simulink model "Slip_Control_codegen"  (R2025b)
settings: Solver=FixedStepDiscrete  StartTime=0.0  StopTime=100  FixedStep=0.003  MaxStep=0.4  RelTol=1e-3  AbsTol=1e-3
model mask{Af=Af, Control=Control, Gr=Gr, L=L, Load_Ref=Load_Ref, MotorT=MotorT, MotorW=MotorW, Slip_Ref=Slip_Ref, Tmax=Tmax, a=a, a_cop=a_cop, cd=cd, g=g, h_CG=h_CG, m=m, ro=ro, rwheel=rwheel, tr=tr, vx_th=vx_th}
model workspace (MAT data in the model file):
  Af = 1.2
  Control.Name = 'SlipControl'
  Control.Steer.Gain.vVehicle.Value = [0 5.26315789474 10.5263157895 15.7894736842 21.0526315789 26.3157894737 31.5789473684 36.8421052632 42.1052631579 47.3684210526 52.6315789474 57.8947368421 63.1578947368 68.4210526316 73.6842105263 78.9473684211 84.2105263158 89.4736842105 94.7368421053 100 180]
  Control.Steer.Gain.vVehicle.Units = 'km/h'
  Control.Steer.Gain.n.Value = [0 -0.3 -0.299810360003 -0.279980668816 -0.23770520484 -0.184653739612 -0.080055401662 0.0617728531856 0.198282548476 0.286925207756 0.3 0.3 0.3 0.3 0.282374573553 0.212225572241 0.119402711766 0.037496894591 9.90231812217e-05 0 0]
  Control.Steer.fActuatorCutoff.Value = 50
  Control.Steer.fActuatorCutoff.Units = 'Hz'
  Control.Steer.Limits.aUpper.Value = 0.174532925199
  Control.Steer.Limits.aUpper.Units = 'rad'
  Control.Steer.Limits.aLower.Value = -0.174532925199
  Control.WheelRad = 0.263
  Control.GearRatio = 5
  Control.MotorTrq = [51.0306904762 51.0306904762 51.0306904762 51.0306904762 51.0306904762 51.0306904762 51.0306904762 51.0306904762 51.0306904762 51.0306904762 51.0306904762 51.0306904762 51.0306904762 51.0306904762 51.0306904762 51.0306904762 51.0306904762 51.0306904762 51.0306904762 51.0306904762 51.0306904762 51.0306904762 51.0306904762 51.0306904762 51.0306904762 51.0306904762 51.0306904762 51.0306904762 51.0306904762 51.0306904762 51.0306904762 51.0306904762 51.0306904762 51.0306904762 51.0306904762 51.0306904762 51.0306904762 44.8436898333 36.8215688219 30.0627288241 25.3370743141 21.0374123095 17.0840324268 13.4184887499 9.99592684833 6.77696534591 3.73957484604]
  Control.MotorW = [0 100 200 300 400 500 600 700 800 900 1000 1100 1200 1300 1400 1500 1600 1700 1800 1900 2000 2100 2200 2300 2400 2500 2600 2700 2800 2900 3000 3100 3200 3300 3400 3500 3600 3700 3800 3900 4000 4100 4200 4300 4400 4500 4600]
  Control.Tmax = 51.0306904762
  Control.RearTrack = 1.248
  Control.FrontTrackToCG = 0.823
  Control.FrontTrackToCoP = 0.8
  Control.FrontalArea = 1.2
  Control.Proportional_P = 1550
  Control.Integral_I = 38025
  Control.Derivative_D = 8
  Control.ActivationVelocity = 0.7
  Control.LiftCoef = -2.15
  Control.GravitationAcc = 9.81
  Control.CGHeight = 0.315
  Control.Wheelbase = 1.575
  Control.Mass = 315
  Control.AirDensity = 1.226
  Control.SlipRef = [0.08; 0.08; 0.152; 0.116; 0.102; 0.096; 0.092; 0.09; 0.09; 0.09; 0.094; 0.098; 0.104; 0.112; 0.126; 0.154; 0.232; 0.1]
  Control.LoadRef = [0; 400; 500; 600; 700; 800; 900; 1000; 1100; 1200; 1300; 1400; 1500; 1600; 1700; 1800; 1900; 2000]
  Gr = 5
  L = 1.578
  Load_Ref = [0; 400; 500; 600; 700; 800; 900; 1000; 1100; 1200; 1300; 1400; 1500; 1600; 1700; 1800; 1900; 2000]
  MotorT = [51.0306904762 51.0306904762 51.0306904762 51.0306904762 51.0306904762 51.0306904762 51.0306904762 51.0306904762 51.0306904762 51.0306904762 51.0306904762 51.0306904762 51.0306904762 51.0306904762 51.0306904762 51.0306904762 51.0306904762 51.0306904762 51.0306904762 51.0306904762 51.0306904762 51.0306904762 51.0306904762 51.0306904762 51.0306904762 51.0306904762 51.0306904762 51.0306904762 51.0306904762 51.0306904762 51.0306904762 51.0306904762 51.0306904762 51.0306904762 51.0306904762 51.0306904762 51.0306904762 44.8436898333 36.8215688219 30.0627288241 25.3370743141 21.0374123095 17.0840324268 13.4184887499 9.99592684833 6.77696534591 3.73957484604]
  MotorW = [0 100 200 300 400 500 600 700 800 900 1000 1100 1200 1300 1400 1500 1600 1700 1800 1900 2000 2100 2200 2300 2400 2500 2600 2700 2800 2900 3000 3100 3200 3300 3400 3500 3600 3700 3800 3900 4000 4100 4200 4300 4400 4500 4600]
  Slip_Ctrl_Kd = Simulink.Parameter
  Slip_Ctrl_Kd.Value = 11
  Slip_Ctrl_Kd.Complexity = 'real'
  Slip_Ctrl_Kd.Dimensions = [1 1]
  Slip_Ctrl_Kd.CoderInfo.StorageClass = 'ImportedExtern'
  Slip_Ctrl_Kd.DataType = 'single'
  Slip_Ctrl_Ki = Simulink.Parameter
  Slip_Ctrl_Ki.Value = 6000
  Slip_Ctrl_Ki.Complexity = 'real'
  Slip_Ctrl_Ki.Dimensions = [1 1]
  Slip_Ctrl_Ki.CoderInfo.StorageClass = 'ImportedExtern'
  Slip_Ctrl_Ki.DataType = 'single'
  Slip_Ctrl_Kn = Simulink.Parameter
  Slip_Ctrl_Kn.Value = 100
  Slip_Ctrl_Kn.Complexity = 'real'
  Slip_Ctrl_Kn.Dimensions = [1 1]
  Slip_Ctrl_Kn.CoderInfo.StorageClass = 'ImportedExtern'
  Slip_Ctrl_Kn.DataType = 'single'
  Slip_Ctrl_Kp = Simulink.Parameter
  Slip_Ctrl_Kp.Value = 800
  Slip_Ctrl_Kp.Complexity = 'real'
  Slip_Ctrl_Kp.Dimensions = [1 1]
  Slip_Ctrl_Kp.CoderInfo.StorageClass = 'ImportedExtern'
  Slip_Ctrl_Kp.DataType = 'single'
  Slip_Ref = [0.08; 0.08; 0.09; 0.095; 0.093; 0.092; 0.091; 0.09; 0.09; 0.09; 0.094; 0.098; 0.104; 0.112; 0.126; 0.154; 0.2; 0.12]
  Tmax = 51.0306904762
  a = 0.8232
  a_cop = 0.707
  cd = -2.15
  g = 9.81
  h_CG = 0.3583
  m = 320
  ro = 1.226
  rwheel = 0.263
  tr = 1.25
  vx_th = 0.7
undefined symbols (not defined in the file or in its folder): dspblkCoreblockFVToolHelper, gcbh
libraries: slpidlib x2
settings Model: TunableVars=Kp  TunableVarsStorageClass=ExportedGlobal  TunableVarsTypeQualifier=const  ParameterArgumentNames=Af,Control,Gr,L,Load_Ref,MotorT,MotorW,Slip_Ref,Tmax,a,a_cop,cd,g,h_CG,m,ro,rwheel,tr,vx_th  Creator=smiller  LastModifiedBy=andrei
settings SolverCC: MaxConsecutiveMinStep=5  AlgebraicLoopSolver=TrustRegion  AutoInsertRateTranBlk=on  InsertRTBMode=Never (minimum delay)  MinimalZcImpactIntegration=on
settings DataIOCC: MaxDataPoints=10000  SaveFormat=StructureWithTime  SaveOutput=off  SignalLogging=off  DSMLogging=off  SaveTime=off  ReturnWorkspaceOutputs=off  SignalLoggingName=logsout_sm_car
settings OptimizationCC: DefaultParameterBehavior=Inlined  UseDivisionForNetSlopeComputation=on  GainParamInheritBuiltInType=on  UseFloatMulNetSlope=on  DefaultUnderspecifiedDataType=single  UseSpecifiedMinMax=on  PassReuseOutputArgsAs=Individual arguments  NoFixptDivByZeroProtection=on  EfficientFloat2IntCast=on  LifeSpan=inf  OptimizeBlockOrder=speed  DifferentSizesBufferReuse=on  EfficientTunableParamExpr=on
settings DebuggingCC: ReadBeforeWriteMsg=EnableAllAsError  WriteAfterWriteMsg=EnableAllAsError  WriteAfterReadMsg=EnableAllAsError  AlgebraicLoopMsg=none  IntegerOverflowMsg=error  ParameterPrecisionLossMsg=none  ParameterTunabilityLossMsg=error  UnconnectedInputMsg=warning  UnconnectedOutputMsg=warning  UnconnectedLineMsg=warning  UniqueDataStoreMsg=error  NonBusSignalsTreatedAsBus=error  SFInvalidInputDataAccessInChartInitDiag=error  SFTransitionOutsideNaturalParentDiag=error  SFUnreachableExecutionPathDiag=error  SFUndirectedBroadcastEventsDiag=error  IntegerSaturationMsg=error  ArithmeticOperatorsInVariantConditions=warning
settings HardwareCC: ProdBitPerPointer=32.0  ProdBitPerSizeT=32.0  ProdBitPerPtrDiffT=32.0  ProdLargestAtomicInteger=Long  ProdLargestAtomicFloat=Double  ProdWordSize=32.0  ProdHWDeviceType=ARM Compatible->ARM Cortex-M
settings ModelReferenceCC: EnableRefExpFcnMdlSchedulingChecks=on
settings SFSimCC: MATLABDynamicMemAlloc=off  CustomCodeUndefinedFunction=UseInterfaceOnly
settings RTWCC: SystemTargetFile=ert.tlc  TemplateMakefile=ert_default_tmf  BuildConfiguration=Faster Runs  GPUComputeCapability=3.5  DLArmComputeVersion=19.05  Description=Embedded Coder
settings CodeAppCC: ForceParamTrailComments=on  IgnoreCustomStorageClasses=off  OperatorAnnotations=on  SimulinkDataObjDesc=on  SFDataObjDesc=on  CustomSymbolStrGlobalVar=rt$N$M  CustomSymbolStrType=$N$M  CustomSymbolStrFcn=$N$M$F  CustomSymbolStrMacro=$N$M  InsertBlockDesc=on
settings ERTTargetCC: ERTCustomFileTemplate=example_file_process.tlc  ERTFilePackagingFormat=CompactWithDataFile  GenerateSampleERTMain=on  IncludeMdlTerminateFcn=off  CombineSignalStateStructs=on  SuppressErrorStatus=on  SupportAbsoluteTime=off  CodeInterfacePackaging=Reusable function  SupportComplex=off
settings SimscapeCC: SimscapeLogType=all  SimscapeLogSimulationStatistics=on  SimscapeLogName=simlog_sm_car  SimscapeLogDataHistory=100000.0  SimscapeOperatingPoint=ssc_op
settings DiagnosticsConfigSet: SimMechanicsConflictingReferenceFrames=none  SimMechanicsRigidlyBoundBlock=none  SimMechanicsUnsatisfiedHighPriorityTargets=error
settings ExplorerConfigSet: InternalSimMechanicsExplorerSettings="<ExplorerConfiguration><canonicalview>default</canonicalview><AnimationSetting><BasePlaybackSpeed>1.0</BasePlaybackSpeed><PlaybackSpeedFactor>1.0</PlaybackSpeedFactor></AnimationSetting><TilePanel><TileInfo><Tiles Columns=\"1\" Count=\"1\" Rows=\"1\"><Column Weight=\"1\"/><Row Weight=\"1\"/><Tile Height=\"1\" Width=\"1\" X=\"0\" Y=\"0\"/></Tiles></TileInfo><SceneInfo><SceneViewer><BGColor><R>1</R><G>1</G><B>1</B></BGColor><Camera><DoPerspective>on</DoPerspective><Position><X>-22.5734563329168161</X><Y>-2.56079992530625722</Y><Z>1.4393604008155032</Z></Position><Center><X>-23.2962680852000119</X><Y>-1.95845679840359432</Y><Z>1.10064823948317181</Z></Center><Up><X>-0.260205889993916473</X><Y>0.216838241661597014</Y><Z>0.940890042335224552</Z></Up><ViewLimDist>1</ViewLimDist><YLim>0.466307658154998694</YLim><XLim>0.489818968650208741</XLim></Camera></SceneViewer></SceneInfo></TilePanel><MechEditorPanel><Cameras><Camera><Id>Camera1</Id><Value><Name>Track FixO FR</Name><NativeCamera><PositionTrackingFeature>Camera_Frames.Frame_FixO_FR.R</PositionTrackingFeature><CenterTrackingFeature>Camera_Frames.Frame_FixO_FR.R</CenterTrackingFeature><UpVectorTrackingFeature>Camera_Frames.Frame_FixO_FR.R</UpVectorTrackingFeature><CenterTrackingOrigin>off</CenterTrackingOrigin><CenterTrackingDirection>+X</CenterTrackingDirection><UpVectorTrackingDirection>+Z</UpVectorTrackingDirection></NativeCamera></Value></Camera><Camera><Id>Camera2</Id><Value><Name>Track FixO Right</Name><NativeCamera><PositionTrackingFeature>Camera_Frames.Frame_FixO_Right.R</PositionTrackingFeature><CenterTrackingFeature>Camera_Frames.Transform_Camera_Ref.F</CenterTrackingFeature><UpVectorTrackingFeature>Camera_Frames.Frame_FixO_Right.R</UpVectorTrackingFeature><CenterTrackingOrigin>off</CenterTrackingOrigin><CenterTrackingDirection>+Y</CenterTrackingDirection><UpVectorTrackingDirection>+Z</UpVectorTrackingDirection></NativeCamera></Value></Camera><Camera><Id>Camera3</Id><Value><Name>Track FixO RR</Name><NativeCamera><PositionTrackingFeature>Camera_Frames.Frame_FixO_RR.R</PositionTrackingFeature><CenterTrackingFeature>Camera_Frames.Frame_FixO_RR.R</CenterTrackingFeature><UpVectorTrackingFeature>Camera_Frames.Frame_FixO_RR.R</UpVectorTrackingFeature><CenterTrackingOrigin>off</CenterTrackingOrigin><CenterTrackingDirection>+X</CenterTrackingDirection><UpVectorTrackingDirection>+Z</UpVectorTrackingDirection></NativeCamera></Value></Camera><Camera><Id>Camera4</Id><Value><Name>Track FixO RL</Name><NativeCamera><PositionTrackingFeature>Camera_Frames.Frame_FixO_RL.R</PositionTrackingFeature><CenterTrackingFeature>Camera_Frames.Frame_FixO_RL.R</CenterTrackingFeature><UpVectorTrackingFeature>Camera_Frames.Frame_FixO_RL.R</UpVectorTrackingFeature><CenterTrackingOrigin>off</CenterTrackingOrigin><CenterTrackingDirection>+X</CenterTrackingDirection><UpVectorTrackingDirection>+Z</UpVectorTrackingDirection></NativeCamera></Value></Camera><Camera><Id>Camera5</Id><Value><Name>Track FixO Left</Name><NativeCamera><PositionTrackingFeature>Camera_Frames.Frame_FixO_Left.R</PositionTrackingFeature><CenterTrackingFeature>Camera_Frames.Transform_Camera_Ref.F</CenterTrackingFeature><UpVectorTrackingFeature>Camera_Frames.Frame_FixO_Left.R</UpVectorTrackingFeature><CenterTrackingOrigin>off</CenterTrackingOrigin><CenterTrackingDirection>-Y</CenterTrackingDirection><UpVectorTrackingDirection>+Z</UpVectorTrackingDirection></NativeCamera></Value></Camera><Camera><Id>Camera6</Id><Value><Name>Track FixO FL</Name><NativeCamera><PositionTrackingFeature>Camera_Frames.Frame_FixO_FL.R</PositionTrackingFeature><CenterTrackingFeature>Camera_Frames.Frame_FixO_FL.R</CenterTrackingFeature><UpVectorTrackingFeature>Camera_Frames.Frame_FixO_FL.R</UpVectorTrackingFeature><CenterTrackingOrigin>off</CenterTrackingOrigin><CenterTrackingDirection>+X</CenterTrackingDirection><UpVectorTrackingDirection>+Z</UpVectorTrackingDirection></NativeCamera></Value></Camera><Camera><Id>Camera7</Id><Value><Name>Track FixO Top</Name><NativeCamera><PositionTrackingFeature>Camera_Frames.Frame_FixO_Top.R</PositionTrackingFeature><CenterTrackingFeature>Camera_Frames.Frame_FixO_Top.R</CenterTrackingFeature><UpVectorTrackingFeature>Camera_Frames.Frame_FixO_Top.R</UpVectorTrackingFeature><CenterTrackingOrigin>off</CenterTrackingOrigin><CenterTrackingDirection>+X</CenterTrackingDirection><UpVectorTrackingDirection>+Z</UpVectorTrackingDirection></NativeCamera></Value></Camera><Camera><Id>Camera8</Id><Value><Name>Track FixO Front</Name><NativeCamera><PositionTrackingFeature>Camera_Frames.Frame_FixO_Front.R</PositionTrackingFeature><CenterTrackingFeature>Camera_Frames.Frame_FixO_Front.R</CenterTrackingFeature><UpVectorTrackingFeature>Camera_Frames.Frame_FixO_Front.R</UpVectorTrackingFeature><CenterTrackingOrigin>off</CenterTrackingOrigin><CenterTrackingDirection>+X</CenterTrackingDirection><UpVectorTrackingDirection>+Z</UpVectorTrackingDirection></NativeCamera></Value></Camera><Camera><Id>Camera9</Id><Value><Name>Track FixO Rear</Name><NativeCamera><PositionTrackingFeature>Camera_Frames.Frame_FixO_Rear.R</PositionTrackingFeature><CenterTrackingFeature>Camera_Frames.Frame_FixO_Rear.R</CenterTrackingFeature><UpVectorTrackingFeature>Camera_Frames.Frame_FixO_Rear.R</UpVectorTrackingFeature><CenterTrackingOrigin>off</CenterTrackingOrigin><CenterTrackingDirection>+X</CenterTrackingDirection><UpVectorTrackingDirection>+Z</UpVectorTrackingDirection></NativeCamera></Value></Camera><Camera><Id>Camera10</Id><Value><Name>Track FR</Name><NativeCamera><PositionTrackingFeature>Camera_Frames.Frame_FR.R</PositionTrackingFeature><CenterTrackingFeature>Camera_Frames.Frame_FR.R</CenterTrackingFeature><UpVectorTrackingFeature>Camera_Frames.Frame_FR.R</UpVectorTrackingFeature><CenterTrackingOrigin>off</CenterTrackingOrigin><CenterTrackingDirection>+X</CenterTrackingDirection><UpVectorTrackingDirection>+Z</UpVectorTrackingDirection></NativeCamera></Value></Camera><Camera><Id>Camera11</Id><Value><Name>Track Right</Name><NativeCamera><PositionTrackingFeature>Camera_Frames.Frame_Right.R</PositionTrackingFeature><CenterTrackingFeature>Camera_Frames.Transform_Camera_Ref.F</CenterTrackingFeature><UpVectorTrackingFeature>Camera_Frames.Frame_Right.R</UpVectorTrackingFeature><CenterTrackingOrigin>off</CenterTrackingOrigin><CenterTrackingDirection>+Y</CenterTrackingDirection><UpVectorTrackingDirection>+Z</UpVectorTrackingDirection></NativeCamera></Value></Camera><Camera><Id>Camera12</Id><Value><Name>Track RR</Name><NativeCamera><PositionTrackingFeature>Camera_Frames.Frame_RR.R</PositionTrackingFeature><CenterTrackingFeature>Camera_Frames.Frame_RR.R</CenterTrackingFeature><UpVectorTrackingFeature>Camera_Frames.Frame_RR.R</UpVectorTrackingFeature><CenterTrackingOrigin>off</CenterTrackingOrigin><CenterTrackingDirection>+X</CenterTrackingDirection><UpVectorTrackingDirection>+Z</UpVectorTrackingDirection></NativeCamera></Value></Camera><Camera><Id>Camera13</Id><Value><Name>Track RL</Name><NativeCamera><PositionTrackingFeature>Camera_Frames.Frame_RL.R</PositionTrackingFeature><CenterTrackingFeature>Camera_Frames.Frame_RL.R</CenterTrackingFeature><UpVectorTrackingFeature>Camera_Frames.Frame_RL.R</UpVectorTrackingFeature><CenterTrackingOrigin>off</CenterTrackingOrigin><CenterTrackingDirection>+X</CenterTrackingDirection><UpVectorTrackingDirection>+Z</UpVectorTrackingDirection></NativeCamera></Value></Camera><Camera><Id>Camera14</Id><Value><Name>Track Left</Name><NativeCamera><PositionTrackingFeature>Camera_Frames.Frame_Left.R</PositionTrackingFeature><CenterTrackingFeature>Camera_Frames.Transform_Camera_Ref.F</CenterTrackingFeature><UpVectorTrackingFeature>Camera_Frames.Frame_Left.R</UpVectorTrackingFeature><CenterTrackingOrigin>off</CenterTrackingOrigin><CenterTrackingDirection>-Y</CenterTrackingDirection><UpVectorTrackingDirection>+Z</UpVectorTrackingDirection></NativeCamera></Value></Camera><Camera><Id>Camera15</Id><Value><Name>Track FL</Name><NativeCamera><PositionTrackingFeature>Camera_Frames.Frame_FL.R</PositionTrackingFeature><CenterTrackingFeature>Camera_Frames.Frame_FL.R</CenterTrackingFeature><UpVectorTrackingFeature>Camera_Frames.Frame_FL.R</UpVectorTrackingFeature><CenterTrackingOrigin>off</CenterTrackingOrigin><CenterTrackingDirection>+X</CenterTrackingDirection><UpVectorTrackingDirection>+Z</UpVectorTrackingDirection></NativeCamera></Value></Camera><Camera><Id>Camera16</Id><Value><Name>Track Top</Name><NativeCamera><PositionTrackingFeature>Camera_Frames.Frame_Top.R</PositionTrackingFeature><CenterTrackingFeature>Camera_Frames.Frame_Top.R</CenterTrackingFeature><UpVectorTrackingFeature>Camera_Frames.Frame_Top.R</UpVectorTrackingFeature><CenterTrackingOrigin>off</CenterTrackingOrigin><CenterTrackingDirection>+X</CenterTrackingDirection><UpVectorTrackingDirection>+Z</UpVectorTrackingDirection></NativeCamera></Value></Camera><Camera><Id>Camera17</Id><Value><Name>Track Front</Name><NativeCamera><PositionTrackingFeature>Camera_Frames.Frame_Front.R</PositionTrackingFeature><CenterTrackingFeature>Camera_Frames.Frame_Front.R</CenterTrackingFeature><UpVectorTrackingFeature>Camera_Frames.Frame_Front.R</UpVectorTrackingFeature><CenterTrackingOrigin>off</CenterTrackingOrigin><CenterTrackingDirection>+X</CenterTrackingDirection><UpVectorTrackingDirection>+Z</UpVectorTrackingDirection></NativeCamera></Value></Camera><Camera><Id>Camera18</Id><Value><Name>Track Rear</Name><NativeCamera><PositionTrackingFeature>Camera_Frames.Frame_Rear.R</PositionTrackingFeature><CenterTrackingFeature>Camera_Frames.Frame_Rear.R</CenterTrackingFeature><UpVectorTrackingFeature>Camera_Frames.Frame_Rear.R</UpVectorTrackingFeature><CenterTrackingOrigin>off</CenterTrackingOrigin><CenterTrackingDirection>+X</CenterTrackingDirection><UpVectorTrackingDirection>+Z</UpVectorTrackingDirection></NativeCamera></Value></Camera><Camera><Id>Camera19</Id><Value><Name>Track SuspF</Name><NativeCamera><PositionTrackingFeature>Camera_Frames.Frame_SuspF.R</PositionTrackingFeature><CenterTrackingFeature>Camera_Frames.Frame_SuspF.R</CenterTrackingFeature><UpVectorTrackingFeature>Camera_Frames.Frame_SuspF.R</UpVectorTrackingFeature><CenterTrackingOrigin>off</CenterTrackingOrigin><CenterTrackingDirection>+X</CenterTrackingDirection><UpVectorTrackingDirection>+Z</UpVectorTrackingDirection></NativeCamera></Value></Camera><Camera><Id>Camera20</Id><Value><Name>Track SuspR</Name><NativeCamera><PositionTrackingFeature>Camera_Frames.Frame_SuspR.R</PositionTrackingFeature><CenterTrackingFeature>Camera_Frames.Frame_SuspR.R</CenterTrackingFeature><UpVectorTrackingFeature>Camera_Frames.Frame_SuspR.R</UpVectorTrackingFeature><CenterTrackingOrigin>off</CenterTrackingOrigin><CenterTrackingDirection>+X</CenterTrackingDirection><UpVectorTrackingDirection>+Z</UpVectorTrackingDirection></NativeCamera></Value></Camera><Camera><Id>Camera21</Id><Value><Name>Track WheelFR</Name><NativeCamera><PositionTrackingFeature>Camera_Frames.Frame_Wheel_FR.R</PositionTrackingFeature><CenterTrackingFeature>Camera_Frames.Frame_Wheel_FR.R</CenterTrackingFeature><UpVectorTrackingFeature>Camera_Frames.Frame_Wheel_FR.R</UpVectorTrackingFeature><CenterTrackingOrigin>off</CenterTrackingOrigin><CenterTrackingDirection>+X</CenterTrackingDirection><UpVectorTrackingDirection>+Z</UpVectorTrackingDirection></NativeCamera></Value></Camera><Camera><Id>Camera22</Id><Value><Name>Track WheelRR</Name><NativeCamera><PositionTrackingFeature>Camera_Frames.Frame_Wheel_RR.R</PositionTrackingFeature><CenterTrackingFeature>Camera_Frames.Frame_Wheel_RR.R</CenterTrackingFeature><UpVectorTrackingFeature>Camera_Frames.Frame_Wheel_RR.R</UpVectorTrackingFeature><CenterTrackingOrigin>off</CenterTrackingOrigin><CenterTrackingDirection>+X</CenterTrackingDirection><UpVectorTrackingDirection>+Z</UpVectorTrackingDirection></NativeCamera></Value></Camera><Camera><Id>Camera23</Id><Value><Name>Track WheelRL</Name><NativeCamera><PositionTrackingFeature>Camera_Frames.Frame_Wheel_RL.R</PositionTrackingFeature><CenterTrackingFeature>Camera_Frames.Frame_Wheel_RL.R</CenterTrackingFeature><UpVectorTrackingFeature>Camera_Frames.Frame_Wheel_RL.R</UpVectorTrackingFeature><CenterTrackingOrigin>off</CenterTrackingOrigin><CenterTrackingDirection>+X</CenterTrackingDirection><UpVectorTrackingDirection>+Z</UpVectorTrackingDirection></NativeCamera></Value></Camera><Camera><Id>Camera24</Id><Value><Name>Track WheelFL</Name><NativeCamera><PositionTrackingFeature>Camera_Frames.Frame_Wheel_FL.R</PositionTrackingFeature><CenterTrackingFeature>Camera_Frames.Frame_Wheel_FL.R</CenterTrackingFeature><UpVectorTrackingFeature>Camera_Frames.Frame_Wheel_FL.R</UpVectorTrackingFeature><CenterTrackingOrigin>off</CenterTrackingOrigin><CenterTrackingDirection>+X</CenterTrackingDirection><UpVectorTrackingDirection>+Z</UpVectorTrackingDirection></NativeCamera></Value></Camera><Camera><Id>Camera25</Id><Value><Name>View Seat FL</Name><NativeCamera><PositionTrackingFeature>Camera_Frames.Frame_View_Seat_FL.R</PositionTrackingFeature><CenterTrackingFeature>Camera_Frames.Frame_View_Seat_FL.R</CenterTrackingFeature><UpVectorTrackingFeature>Camera_Frames.Frame_View_Seat_FL.R</UpVectorTrackingFeature><CenterTrackingOrigin>off</CenterTrackingOrigin><CenterTrackingDirection>+X</CenterTrackingDirection><UpVectorTrackingDirection>+Z</UpVectorTrackingDirection></NativeCamera></Value></Camera><Camera><Id>Camera26</Id><Value><Name>View Seat FR</Name><NativeCamera><PositionTrackingFeature>Camera_Frames.Frame_View_Seat_FR.R</PositionTrackingFeature><CenterTrackingFeature>Camera_Frames.Frame_View_Seat_FR.R</CenterTrackingFeature><UpVectorTrackingFeature>Camera_Frames.Frame_View_Seat_FR.R</UpVectorTrackingFeature><CenterTrackingOrigin>off</CenterTrackingOrigin><CenterTrackingDirection>+X</CenterTrackingDirection><UpVectorTrackingDirection>+Z</UpVectorTrackingDirection></NativeCamera></Value></Camera><Camera><Id>Camera27</Id><Value><Name>View Susp FR</Name><NativeCamera><PositionTrackingFeature>Camera_Frames.Frame_View_Susp_FR.R</PositionTrackingFeature><CenterTrackingFeature>Camera_Frames.Frame_View_Susp_FR.R</CenterTrackingFeature><UpVectorTrackingFeature>Camera_Frames.Frame_View_Susp_FR.R</UpVectorTrackingFeature><CenterTrackingOrigin>off</CenterTrackingOrigin><CenterTrackingDirection>+X</CenterTrackingDirection><UpVectorTrackingDirection>+Z</UpVectorTrackingDirection></NativeCamera></Value></Camera><Camera><Id>Camera28</Id><Value><Name>View Susp RR</Name><NativeCamera><PositionTrackingFeature>Camera_Frames.Frame_View_Susp_RR.R</PositionTrackingFeature><CenterTrackingFeature>Camera_Frames.Frame_View_Susp_RR.R</CenterTrackingFeature><UpVectorTrackingFeature>Camera_Frames.Frame_View_Susp_RR.R</UpVectorTrackingFeature><CenterTrackingOrigin>off</CenterTrackingOrigin><CenterTrackingDirection>+X</CenterTrackingDirection><UpVectorTrackingDirection>+Z</UpVectorTrackingDirection></NativeCamera></Value></Camera><Camera><Id>Camera29</Id><Value><Name>View Susp RL</Name><NativeCamera><PositionTrackingFeature>Camera_Frames.Frame_View_Susp_RL.R</PositionTrackingFeature><CenterTrackingFeature>Camera_Frames.Frame_View_Susp_RL.R</CenterTrackingFeature><UpVectorTrackingFeature>Camera_Frames.Frame_View_Susp_RL.R</UpVectorTrackingFeature><CenterTrackingOrigin>off</CenterTrackingOrigin><CenterTrackingDirection>+X</CenterTrackingDirection><UpVectorTrackingDirection>+Z</UpVectorTrackingDirection></NativeCamera></Value></Camera><Camera><Id>Camera30</Id><Value><Name>View Susp FL</Name><NativeCamera><PositionTrackingFeature>Camera_Frames.Frame_View_Susp_FL.R</PositionTrackingFeature><CenterTrackingFeature>Camera_Frames.Frame_View_Susp_FL.R</CenterTrackingFeature><UpVectorTrackingFeature>Camera_Frames.Frame_View_Susp_FL.R</UpVectorTrackingFeature><CenterTrackingOrigin>off</CenterTrackingOrigin><CenterTrackingDirection>+X</CenterTrackingDirection><UpVectorTrackingDirection>+Z</UpVectorTrackingDirection></NativeCamera></Value></Camera><Camera><Id>Camera31</Id><Value><Name>Dolly Camera</Name><NativeCamera><PositionTrackingFeature>Camera_Frames.Frame_Dolly.R</PositionTrackingFeature><CenterTrackingFeature>Camera_Frames.Frame_Dolly.R</CenterTrackingFeature><UpVectorTrackingFeature>Camera_Frames.Frame_Dolly.R</UpVectorTrackingFeature><CenterTrackingOrigin>off</CenterTrackingOrigin><CenterTrackingDirection>+X</CenterTrackingDirection><UpVectorTrackingDirection>+Z</UpVectorTrackingDirection></NativeCamera></Value></Camera><Camera><Id>Camera32</Id><Value><Name>Track Dolly Camera</Name><NativeCamera><PositionTrackingFeature>Camera_Frames.Frame_Dolly.R</PositionTrackingFeature><CenterTrackingFeature>Camera_Frames.Transform_Camera_Ref.F</CenterTrackingFeature><UpVectorTrackingFeature>Camera_Frames.World_Frame.W</UpVectorTrackingFeature><CenterTrackingOrigin>on</CenterTrackingOrigin><UpVectorTrackingDirection>+Z</UpVectorTrackingDirection></NativeCamera></Value></Camera></Cameras><GfxPanelCameraMap><MapElement CameraMLId=\"Camera1\" GfxPanelIndex=\"0\"/></GfxPanelCameraMap><VideoCreator><PlaybackSpeedRatio>1.0</PlaybackSpeedRatio><FrameRate>30</FrameRate><VideoFormat>MPEG-4</VideoFormat><FrameSize>[800 450]</FrameSize></VideoCreator></MechEditorPanel></ExplorerConfiguration>"

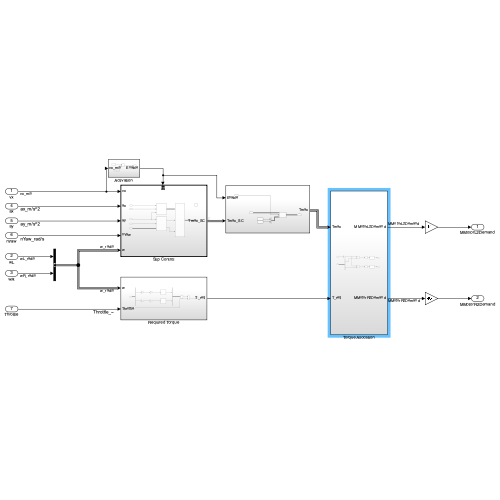
[thumbnail: Simulink's stored preview of the top-level diagram]
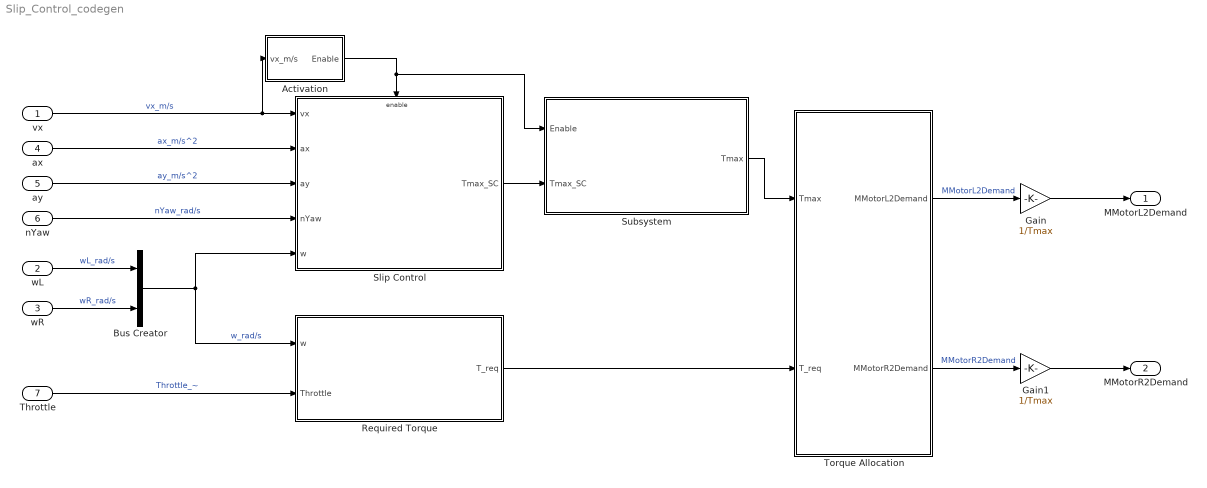
== system Slip_Control_codegen ==
  vx : Inport  OutDataTypeStr=single  PortDimensions=1  SampleTime=0.003  Interpolate=off
  wL : Inport  Port=2  OutDataTypeStr=single  PortDimensions=1  SampleTime=0.003
  wR : Inport  Port=3  OutDataTypeStr=single  PortDimensions=1  SampleTime=0.003
  ax : Inport  Port=4  OutDataTypeStr=single  PortDimensions=1  SampleTime=0.003
  ay : Inport  Port=5  OutDataTypeStr=single  PortDimensions=1  SampleTime=0.003
  nYaw : Inport  Port=6  OutDataTypeStr=single  PortDimensions=1  SampleTime=0.003
  Throttle : Inport  Port=7  OutDataTypeStr=single  PortDimensions=1  SampleTime=0.003
  Activation : Subsystem
  Bus Creator : BusCreator  Inputs=2
  Gain : Gain  Gain=1/Tmax  ParamDataTypeStr=single  OutDataTypeStr=single
  Gain1 : Gain  Gain=1/Tmax  ParamDataTypeStr=single  OutDataTypeStr=single
  Required Torque : Subsystem
  Slip Control : Subsystem
  Subsystem : Subsystem
  Torque Allocation : Subsystem
  MMotorL2Demand : Outport  OutDataTypeStr=single  PortDimensions=1  SampleTime=0.003
  MMotorR2Demand : Outport  Port=2  OutDataTypeStr=single  PortDimensions=1  SampleTime=0.003
  wires:
  Gain1/1 -> MMotorR2Demand/1
  Throttle/1 -> Required Torque/2(Throttle)  "Throttle_~"
  Torque Allocation/1(MMotorL2Demand) -> Gain/1  "MMotorL2Demand"
  Required Torque/1(T_req) -> Torque Allocation/2(T_req)
  wL/1 -> Bus Creator/1  "wL_rad/s"
  Bus Creator/1 -> Slip Control/5(w), Required Torque/1(w)  "w_rad/s"
  wR/1 -> Bus Creator/2  "wR_rad/s"
  Torque Allocation/2(MMotorR2Demand) -> Gain1/1  "MMotorR2Demand"
  Gain/1 -> MMotorL2Demand/1
  ax/1 -> Slip Control/2(ax)  "ax_m/s^2"
  ay/1 -> Slip Control/3(ay)  "ay_m/s^2"
  vx/1 -> Activation/1(vx_m/s), Slip Control/1(vx)  "vx_m/s"
  nYaw/1 -> Slip Control/4(nYaw)  "nYaw_rad/s"
  Activation/1(Enable) -> Subsystem/1(Enable), Slip Control/Enable
  Slip Control/1(Tmax_SC) -> Subsystem/2(Tmax_SC)
  Subsystem/1(Tmax) -> Torque Allocation/1(Tmax)

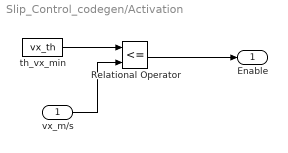
== system Slip_Control_codegen/Activation ==
  vx_m/s : Inport
  Relational Operator : RelationalOperator  Operator=<=  OutDataTypeStr=boolean  RndMeth=Simplest  InputSameDT=off
  th_vx_min : Constant  Value=vx_th  OutDataTypeStr=single
  Enable : Outport
  wires:
  Relational Operator/1 -> Enable/1
  vx_m/s/1 -> Relational Operator/2
  th_vx_min/1 -> Relational Operator/1

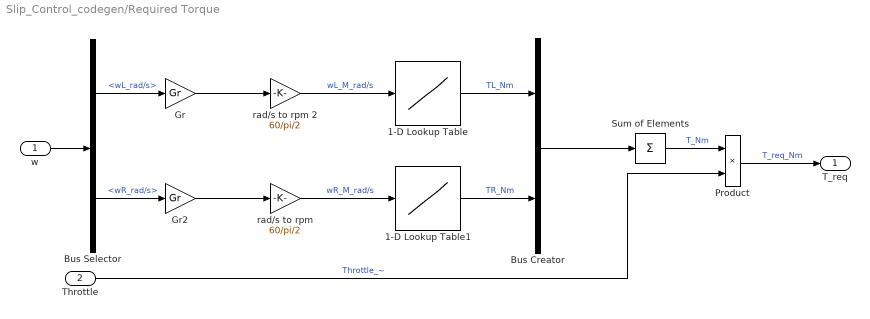
== system Slip_Control_codegen/Required Torque ==
  w : Inport  SampleTime=0.003
  Throttle : Inport  Port=2  OutDataTypeStr=single  PortDimensions=1  SampleTime=0.003
  1-D Lookup Table : Lookup_n-D  NumberOfTableDimensions=1  BreakpointsForDimension1=MotorW  Table=MotorT  InternalRulePriority=Speed  RndMeth=Simplest
  1-D Lookup Table1 : Lookup_n-D  NumberOfTableDimensions=1  BreakpointsForDimension1=MotorW  Table=MotorT  InternalRulePriority=Speed  RndMeth=Simplest
  Bus Creator : BusCreator  Inputs=2
  Bus Selector : BusSelector  OutputSignals=wL_rad/s,wR_rad/s
  Gr : Gain  Gain=Gr
  Gr2 : Gain  Gain=Gr
  Product : Product
  Sum of Elements : Sum  Inputs=+
  rad/s to rpm : Gain  Gain=60/pi/2
  rad/s to rpm 2 : Gain  Gain=60/pi/2
  T_req : Outport  OutDataTypeStr=single  PortDimensions=1  SampleTime=0.003
  wires:
  w/1 -> Bus Selector/1
  Sum of Elements/1 -> Product/1  "T_Nm"
  1-D Lookup Table1/1 -> Bus Creator/2  "TR_Nm"
  Throttle/1 -> Product/2  "Throttle_~"
  rad/s to rpm/1 -> 1-D Lookup Table1/1  "wR_M_rad/s"
  Bus Selector/1 -> Gr/1  "<wL_rad/s>"
  Product/1 -> T_req/1  "T_req_Nm"
  Bus Selector/2 -> Gr2/1  "<wR_rad/s>"
  rad/s to rpm 2/1 -> 1-D Lookup Table/1  "wL_M_rad/s"
  1-D Lookup Table/1 -> Bus Creator/1  "TL_Nm"
  Bus Creator/1 -> Sum of Elements/1
  Gr/1 -> rad/s to rpm 2/1
  Gr2/1 -> rad/s to rpm/1

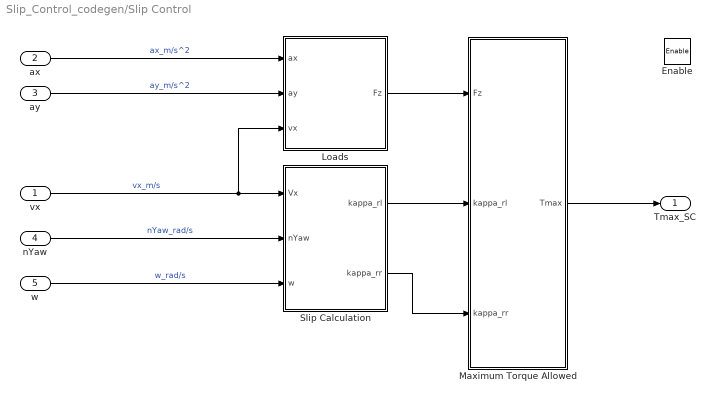
== system Slip_Control_codegen/Slip Control ==
  vx : Inport  OutDataTypeStr=single  PortDimensions=1  SampleTime=0.003
  ax : Inport  Port=2  OutDataTypeStr=single  PortDimensions=1  SampleTime=0.003
  ay : Inport  Port=3  OutDataTypeStr=single  PortDimensions=1  SampleTime=0.003
  nYaw : Inport  Port=4  OutDataTypeStr=single  PortDimensions=1  SampleTime=0.003
  w : Inport  Port=5  SampleTime=0.003
  Enable : EnablePort
  Loads : Subsystem
  Maximum Torque Allowed : Subsystem
  Slip Calculation : Subsystem
  Tmax_SC : Outport  SampleTime=0.003
  wires:
  Slip Calculation/1(kappa_rl) -> Maximum Torque Allowed/2(kappa_rl)
  Maximum Torque Allowed/1(Tmax) -> Tmax_SC/1
  vx/1 -> Slip Calculation/1(Vx), Loads/3(vx)  "vx_m/s"
  Slip Calculation/2(kappa_rr) -> Maximum Torque Allowed/3(kappa_rr)
  ay/1 -> Loads/2(ay)  "ay_m/s^2"
  Loads/1(Fz) -> Maximum Torque Allowed/1(Fz)
  ax/1 -> Loads/1(ax)  "ax_m/s^2"
  nYaw/1 -> Slip Calculation/2(nYaw)  "nYaw_rad/s"
  w/1 -> Slip Calculation/3(w)  "w_rad/s"

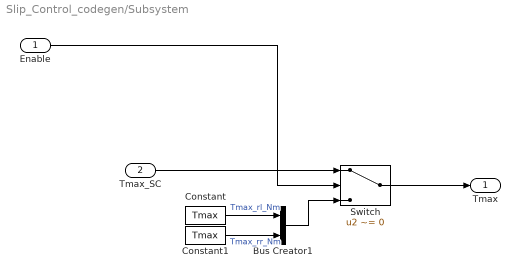
== system Slip_Control_codegen/Subsystem ==
  Enable : Inport
  Tmax_SC : Inport  Port=2
  Bus Creator1 : BusCreator  Inputs=2
  Constant : Constant  Value=Tmax  OutDataTypeStr=single
  Constant1 : Constant  Value=Tmax  OutDataTypeStr=single
  Switch : Switch  Criteria=u2 ~= 0  SaturateOnIntegerOverflow=off  InputSameDT=off
  Tmax : Outport
  wires:
  Tmax_SC/1 -> Switch/1
  Constant1/1 -> Bus Creator1/2  "Tmax_rr_Nm"
  Switch/1 -> Tmax/1
  Enable/1 -> Switch/2
  Bus Creator1/1 -> Switch/3
  Constant/1 -> Bus Creator1/1  "Tmax_rl_Nm"

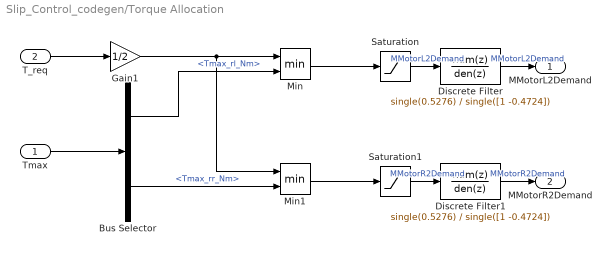
== system Slip_Control_codegen/Torque Allocation ==
  Tmax : Inport  OutDataTypeStr=single  SampleTime=0.003
  T_req : Inport  Port=2  OutDataTypeStr=single  PortDimensions=1  SampleTime=0.003
  Bus Selector : BusSelector  OutputSignals=Tmax_rl_Nm,Tmax_rr_Nm
  Discrete Filter : DiscreteFilter  LoadFcn=dspblkCoreblockFVToolHelper(gcbh,'load');  Numerator=single(0.5276)  Denominator=single([1 -0.4724])  InitialStates=single(0)  SampleTime=0.003
      settings: CopyFcn=dspblkCoreblockFVToolHelper(gcbh,'copy');  DeleteFcn=dspblkCoreblockFVToolHelper(gcbh,'close');  ModelCloseFcn=dspblkCoreblockFVToolHelper(gcbh,'close');  PreSaveFcn=dspblkCoreblockFVToolHelper(gcbh,'presave');  PostSaveFcn=dspblkCoreblockFVToolHelper(gcbh,'postsave');  CloseFcn=dspblkCoreblockFVToolHelper(gcbh,'close');
  Discrete Filter1 : DiscreteFilter  LoadFcn=dspblkCoreblockFVToolHelper(gcbh,'load');  Numerator=single(0.5276)  Denominator=single([1 -0.4724])  InitialStates=single(0)  SampleTime=0.003
      settings: CopyFcn=dspblkCoreblockFVToolHelper(gcbh,'copy');  DeleteFcn=dspblkCoreblockFVToolHelper(gcbh,'close');  ModelCloseFcn=dspblkCoreblockFVToolHelper(gcbh,'close');  PreSaveFcn=dspblkCoreblockFVToolHelper(gcbh,'presave');  PostSaveFcn=dspblkCoreblockFVToolHelper(gcbh,'postsave');  CloseFcn=dspblkCoreblockFVToolHelper(gcbh,'close');
  Gain1 : Gain  Gain=1/2  ParamDataTypeStr=single  OutDataTypeStr=single
  Min : MinMax  Inputs=2  OutDataTypeStr=single
  Min1 : MinMax  Inputs=2  OutDataTypeStr=single
  Saturation : Saturate  UpperLimit=Tmax  LowerLimit=0  OutDataTypeStr=single
  Saturation1 : Saturate  UpperLimit=Tmax  LowerLimit=0  OutDataTypeStr=single
  MMotorL2Demand : Outport  OutDataTypeStr=single  PortDimensions=1  SampleTime=0.003
  MMotorR2Demand : Outport  Port=2  OutDataTypeStr=single  PortDimensions=1  SampleTime=0.003
  wires:
  Bus Selector/2 -> Min1/2  "<Tmax_rr_Nm>"
  T_req/1 -> Gain1/1
  Gain1/1 -> Min1/1, Min/1
  Min1/1 -> Saturation1/1
  Min/1 -> Saturation/1
  Tmax/1 -> Bus Selector/1
  Bus Selector/1 -> Min/2  "<Tmax_rl_Nm>"
  Saturation/1 -> Discrete Filter/1  "MMotorL2Demand"
  Discrete Filter/1 -> MMotorL2Demand/1  "MMotorL2Demand"
  Saturation1/1 -> Discrete Filter1/1  "MMotorR2Demand"
  Discrete Filter1/1 -> MMotorR2Demand/1  "MMotorR2Demand"

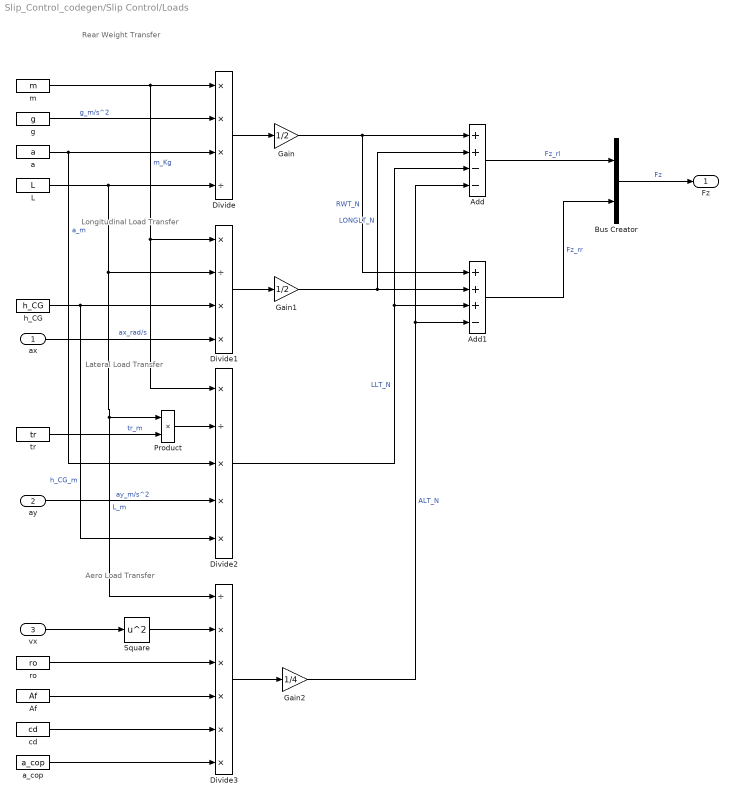
== system Slip_Control_codegen/Slip Control/Loads ==
  note: Rear Weight Transfer
  note: Longitudinal Load Transfer
  note: Lateral Load Transfer
  note: Aero Load Transfer
  ax : Inport  OutDataTypeStr=single  PortDimensions=1  SampleTime=0.003
  ay : Inport  Port=2  OutDataTypeStr=single  PortDimensions=1  SampleTime=0.003
  vx : Inport  Port=3  OutDataTypeStr=single  PortDimensions=1  SampleTime=0.003
  Add : Sum  Inputs=++--  OutDataTypeStr=single  AccumDataTypeStr=single
  Add1 : Sum  Inputs=+++-  OutDataTypeStr=single  AccumDataTypeStr=single
  Af : Constant  Value=Af  OutDataTypeStr=single
  Bus Creator : BusCreator  Inputs=2
  Divide : Product  Inputs=***/  OutDataTypeStr=single
  Divide1 : Product  Inputs=*/**  OutDataTypeStr=single
  Divide2 : Product  Inputs=*/***  OutDataTypeStr=single
  Divide3 : Product  Inputs=/*****  OutDataTypeStr=single
  Gain : Gain  Gain=1/2  ParamDataTypeStr=single  OutDataTypeStr=single
  Gain1 : Gain  Gain=1/2  ParamDataTypeStr=single  OutDataTypeStr=single
  Gain2 : Gain  Gain=1/4  ParamDataTypeStr=single  OutDataTypeStr=single
  L : Constant  Value=L  OutDataTypeStr=single
  Product : Product  OutDataTypeStr=single
  Square : Math  Operator=square  OutDataTypeStr=single
  a : Constant  Value=a  OutDataTypeStr=single
  a_cop : Constant  Value=a_cop  OutDataTypeStr=single
  cd : Constant  Value=cd  OutDataTypeStr=single
  g : Constant  Value=g  OutDataTypeStr=single
  h_CG : Constant  Value=h_CG  OutDataTypeStr=single
  m : Constant  Value=m  OutDataTypeStr=single
  ro : Constant  Value=ro  OutDataTypeStr=single
  tr : Constant  Value=tr  OutDataTypeStr=single
  Fz : Outport  SampleTime=0.003
  wires:
  a_cop/1 -> Divide3/6
  cd/1 -> Divide3/5
  Af/1 -> Divide3/4
  ro/1 -> Divide3/3
  Divide3/1 -> Gain2/1
  Bus Creator/1 -> Fz/1  "Fz"
  Add1/1 -> Bus Creator/2  "Fz_rr"
  Add/1 -> Bus Creator/1  "Fz_rl"
  Divide2/1 -> Add1/3, Add/3  "LLT_N"
  tr/1 -> Product/2  "tr_m"
  ay/1 -> Divide2/4  "ay_m/s^2"
  Gain1/1 -> Add1/2, Add/2  "LONGLT_N"
  Divide1/1 -> Gain1/1
  ax/1 -> Divide1/4  "ax_rad/s"
  h_CG/1 -> Divide1/3, Divide2/5  "h_CG_m"
  Gain2/1 -> Add1/4, Add/4  "ALT_N"
  Gain/1 -> Add1/1, Add/1  "RWT_N"
  Square/1 -> Divide3/2
  vx/1 -> Square/1
  Divide/1 -> Gain/1
  L/1 -> Divide/4, Divide1/2, Divide3/1, Product/1  "L_m"
  a/1 -> Divide2/3, Divide/3  "a_m"
  g/1 -> Divide/2  "g_m/s^2"
  m/1 -> Divide2/1, Divide1/1, Divide/1  "m_Kg"
  Product/1 -> Divide2/2

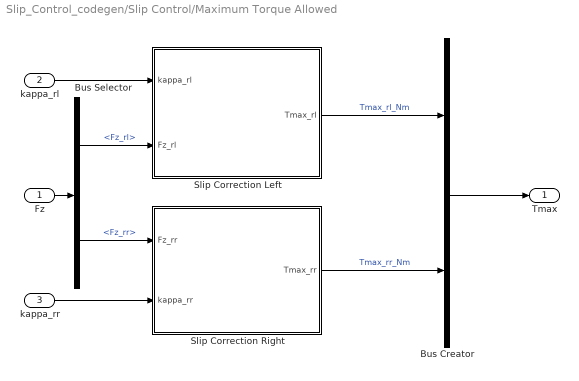
== system Slip_Control_codegen/Slip Control/Maximum Torque Allowed ==
  Fz : Inport  SampleTime=0.003
  kappa_rl : Inport  Port=2  OutDataTypeStr=single  PortDimensions=1  SampleTime=0.003
  kappa_rr : Inport  Port=3  OutDataTypeStr=single  PortDimensions=1  SampleTime=0.003
  Bus Creator : BusCreator  Inputs=2
  Bus Selector : BusSelector  OutputSignals=Fz_rl,Fz_rr
  Slip Correction Left : Subsystem
  Slip Correction Right : Subsystem
  Tmax : Outport  SampleTime=0.003
  wires:
  Bus Creator/1 -> Tmax/1
  Bus Selector/2 -> Slip Correction Right/1(Fz_rr)  "<Fz_rr>"
  Bus Selector/1 -> Slip Correction Left/2(Fz_rl)  "<Fz_rl>"
  Fz/1 -> Bus Selector/1
  kappa_rr/1 -> Slip Correction Right/2(kappa_rr)
  kappa_rl/1 -> Slip Correction Left/1(kappa_rl)
  Slip Correction Left/1(Tmax_rl) -> Bus Creator/1  "Tmax_rl_Nm"
  Slip Correction Right/1(Tmax_rr) -> Bus Creator/2  "Tmax_rr_Nm"

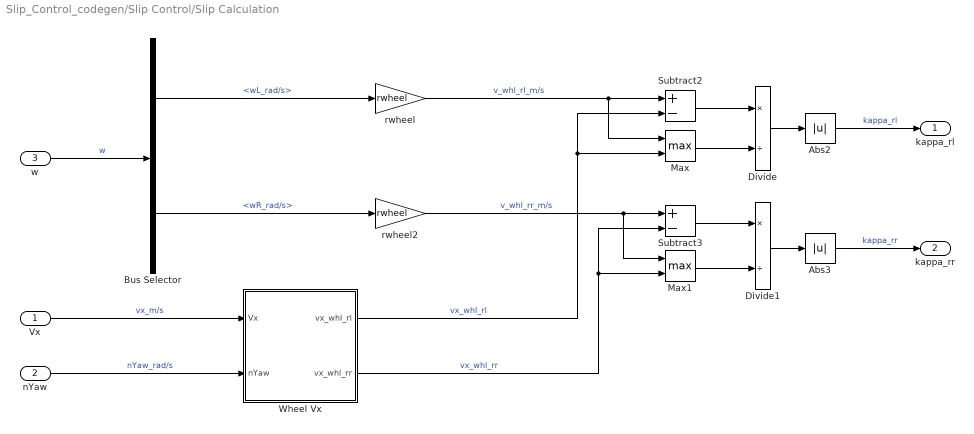
== system Slip_Control_codegen/Slip Control/Slip Calculation ==
  Vx : Inport  OutDataTypeStr=single  PortDimensions=1  SampleTime=0.003
  nYaw : Inport  Port=2  OutDataTypeStr=single  PortDimensions=1  SampleTime=0.003
  w : Inport  Port=3  SampleTime=0.003
  Abs2 : Abs  SaturateOnIntegerOverflow=off
  Abs3 : Abs  SaturateOnIntegerOverflow=off
  Bus Selector : BusSelector  OutputSignals=wL_rad/s,wR_rad/s
  Divide : Product  Inputs=*/
  Divide1 : Product  Inputs=*/
  Max : MinMax  Function=max  Inputs=2
  Max1 : MinMax  Function=max  Inputs=2
  Subtract2 : Sum  Inputs=+-
  Subtract3 : Sum  Inputs=+-
  Wheel Vx : Subsystem
  rwheel : Gain  Gain=rwheel
  rwheel2 : Gain  Gain=rwheel
  kappa_rl : Outport  OutDataTypeStr=single  PortDimensions=1  SampleTime=0.003
  kappa_rr : Outport  Port=2  OutDataTypeStr=single  PortDimensions=1  SampleTime=0.003
  wires:
  Max1/1 -> Divide1/2
  Divide1/1 -> Abs3/1
  Max/1 -> Divide/2
  Divide/1 -> Abs2/1
  Subtract3/1 -> Divide1/1
  Wheel Vx/2(vx_whl_rr) -> Max1/2, Subtract3/2  "vx_whl_rr"
  Subtract2/1 -> Divide/1
  Abs2/1 -> kappa_rl/1  "kappa_rl"
  Wheel Vx/1(vx_whl_rl) -> Max/2, Subtract2/2  "vx_whl_rl"
  Abs3/1 -> kappa_rr/1  "kappa_rr"
  nYaw/1 -> Wheel Vx/2(nYaw)  "nYaw_rad/s"
  rwheel2/1 -> Subtract3/1, Max1/1  "v_whl_rr_m/s"
  rwheel/1 -> Subtract2/1, Max/1  "v_whl_rl_m/s"
  w/1 -> Bus Selector/1  "w"
  Vx/1 -> Wheel Vx/1(Vx)  "vx_m/s"
  Bus Selector/2 -> rwheel2/1  "<wR_rad/s>"
  Bus Selector/1 -> rwheel/1  "<wL_rad/s>"

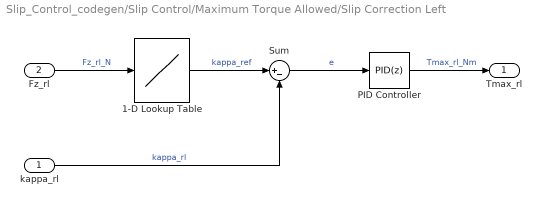
== system Slip_Control_codegen/Slip Control/Maximum Torque Allowed/Slip Correction Left ==
  kappa_rl : Inport  OutDataTypeStr=single  PortDimensions=1  SampleTime=0.003
  Fz_rl : Inport  Port=2  OutDataTypeStr=single  PortDimensions=1  SampleTime=0.003
  1-D Lookup Table : Lookup_n-D  NumberOfTableDimensions=1  BreakpointsForDimension1=Load_Ref  Table=Slip_Ref  ExtrapMethod=Clip  UseLastTableValue=on  InternalRulePriority=Speed  RndMeth=Simplest
  PID Controller : slpidlib/PID Controller  Controller=PID  Form=Parallel  TimeDomain=Discrete-time  UseExternalTs=off  SampleTime=0.003  IntegratorMethod=Forward Euler  FilterMethod=Forward Euler  ControllerParametersSource=internal  P=Slip_Ctrl_Kp  I=Slip_Ctrl_Ki  UseKiTs=off  D=Slip_Ctrl_Kd  UseExternalDerivativeSource=off  N=Slip_Ctrl_Kn  UseFilter=on  TunerSelectOption=Transfer Function Based (PID Tuner App)  InitialConditionSource=internal  InitialConditionForIntegrator=Tmax  InitialConditionForFilter=0  DifferentiatorICPrevScaledInput=Tmax  ExternalReset=none  TrackingMode=off  Kt=1  LimitOutput=on  SatLimitsSource=internal  UpperSaturationLimit=Tmax  LowerSaturationLimit=0  LinearizeAsGain=on  AntiWindupMode=clamping  Kb=1  LimitIntegrator=off  UpperIntegratorSaturationLimit=inf  LowerIntegratorSaturationLimit=-inf  POutMin=[]  POutMax=[]  IOutMin=[]  IOutMax=[]  DOutMin=[]  DOutMax=[]  NOutMin=[]  NOutMax=[]  SumOutMin=[]  SumOutMax=[]  SaturationOutMin=[]  SaturationOutMax=[]  PParamMin=[]  PParamMax=[]  IParamMin=[]  IParamMax=[]  DParamMin=[]  DParamMax=[]  NParamMin=[]  NParamMax=[]  KbParamMin=[]  KbParamMax=[]  KtParamMin=[]  KtParamMax=[]  KbOutMin=[]  KbOutMax=[]  KtOutMin=[]  KtOutMax=[]  IntegratorOutMin=[]  IntegratorOutMax=[]  FilterOutMin=[]  FilterOutMax=[]  SumI1OutMin=[]  SumI1OutMax=[]  SumI2OutMin=[]  SumI2OutMax=[]  SumI3OutMin=[]  SumI3OutMax=[]  SumI4OutMin=[]  SumI4OutMax=[]  SumDOutMin=[]  SumDOutMax=[]  DifferentiatorOutMin=[]  DifferentiatorOutMax=[]  FilterDiffOutCoefMin=[]  FilterDiffOutCoefMax=[]  ReciprocalOutMin=[]  ReciprocalOutMax=[]  SumDenOutMin=[]  SumDenOutMax=[]  SumNumOutMin=[]  SumNumOutMax=[]  DivideOutMin=[]  DivideOutMax=[]  UdiffTsProdOutMin=[]  UdiffTsProdOutMax=[]  NTsProdOutMin=[]  NTsProdOutMax=[]  UintegralTsProdOutMin=[]  UintegralTsProdOutMax=[]  UngainTsProdOutMin=[]  UngainTsProdOutMax=[]  ClampingZeroOutDataTypeStr=Inherit: Inherit via back propagation  ClampingZeroOutMin=[]  ClampingZeroOutMax=[]  FilterDenConstantOutDataTypeStr=Inherit: Inherit via back propagation  FilterDenConstantOutMin=[]  FilterDenConstantOutMax=[]  PCopyOutDataTypeStr=Inherit: Inherit via back propagation  PCopyOutMin=[]  PCopyOutMax=[]  NCopyOutDataTypeStr=Inherit: Inherit via back propagation  NCopyOutMin=[]  NCopyOutMax=[]  IntegratorContinuousStateAttributes=''  IntegratorStateMustResolveToSignalObject=off  IntegratorRTWStateStorageClass=Auto  FilterContinuousStateAttributes=''  FilterStateMustResolveToSignalObject=off  FilterRTWStateStorageClass=Auto  ParallelPVariant=InternalParameters  IdealPVariant=Disabled  IVariant=InternalParameters  DVariant=InternalParameters  IntegratorVariant=Discrete  SatVariant=Enabled  AWVariant=DiscClampingParallel  PCopyVariant=Disabled  TRVariant=Disabled  FdbkBlocksVariant=Forward  IdealPFdbkVariant=Disabled  SatFdbkVariant=Disabled  DerivativeFilterVariant=ForwardEulerFilter  NVariant=InternalParameters  NCopyVariant=Disabled  FilterICVariant=InternalICsFilter  IntegratorICVariant=InternalICs  ExternalResetVariant=Disabled  TRSumVariant=Passthrough  SumFdbkVariant=Disabled  SumVariant=Sum_PID  TsampFilterVariant=InternalTs  TsampNgainVariant=Passthrough  TsampIntegralVariant=Disabled_SignalSpec  ExternalSaturationOutDataTypeStr=Inherit: Same as second input  DerivativeSourceVariant=ErrorSignal  PreIntVariant=InternalPreInt
  Sum : Sum  Inputs=|+-
  Tmax_rl : Outport  OutDataTypeStr=single  PortDimensions=1  SampleTime=0.003
  wires:
  PID Controller/1 -> Tmax_rl/1  "Tmax_rl_Nm"
  Fz_rl/1 -> 1-D Lookup Table/1  "Fz_rl_N"
  Sum/1 -> PID Controller/1  "e"
  1-D Lookup Table/1 -> Sum/1  "kappa_ref"
  kappa_rl/1 -> Sum/2  "kappa_rl"

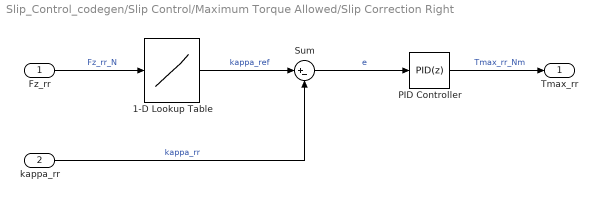
== system Slip_Control_codegen/Slip Control/Maximum Torque Allowed/Slip Correction Right ==
  Fz_rr : Inport  OutDataTypeStr=single  PortDimensions=1  SampleTime=0.003
  kappa_rr : Inport  Port=2  OutDataTypeStr=single  PortDimensions=1  SampleTime=0.003
  1-D Lookup Table : Lookup_n-D  NumberOfTableDimensions=1  BreakpointsForDimension1=Load_Ref  Table=Slip_Ref  ExtrapMethod=Clip  UseLastTableValue=on  InternalRulePriority=Speed  RndMeth=Simplest
  PID Controller : slpidlib/PID Controller  Controller=PID  Form=Parallel  TimeDomain=Discrete-time  UseExternalTs=off  SampleTime=0.003  IntegratorMethod=Forward Euler  FilterMethod=Forward Euler  ControllerParametersSource=internal  P=Slip_Ctrl_Kp  I=Slip_Ctrl_Ki  UseKiTs=off  D=Slip_Ctrl_Kd  UseExternalDerivativeSource=off  N=Slip_Ctrl_Kn  UseFilter=on  TunerSelectOption=Transfer Function Based (PID Tuner App)  InitialConditionSource=internal  InitialConditionForIntegrator=Tmax  InitialConditionForFilter=0  DifferentiatorICPrevScaledInput=Tmax  ExternalReset=none  TrackingMode=off  Kt=1  LimitOutput=on  SatLimitsSource=internal  UpperSaturationLimit=Tmax  LowerSaturationLimit=0  LinearizeAsGain=on  AntiWindupMode=clamping  Kb=1  LimitIntegrator=off  UpperIntegratorSaturationLimit=inf  LowerIntegratorSaturationLimit=-inf  POutMin=[]  POutMax=[]  IOutMin=[]  IOutMax=[]  DOutMin=[]  DOutMax=[]  NOutMin=[]  NOutMax=[]  SumOutMin=[]  SumOutMax=[]  SaturationOutMin=[]  SaturationOutMax=[]  PParamMin=[]  PParamMax=[]  IParamMin=[]  IParamMax=[]  DParamMin=[]  DParamMax=[]  NParamMin=[]  NParamMax=[]  KbParamMin=[]  KbParamMax=[]  KtParamMin=[]  KtParamMax=[]  KbOutMin=[]  KbOutMax=[]  KtOutMin=[]  KtOutMax=[]  IntegratorOutMin=[]  IntegratorOutMax=[]  FilterOutMin=[]  FilterOutMax=[]  SumI1OutMin=[]  SumI1OutMax=[]  SumI2OutMin=[]  SumI2OutMax=[]  SumI3OutMin=[]  SumI3OutMax=[]  SumI4OutMin=[]  SumI4OutMax=[]  SumDOutMin=[]  SumDOutMax=[]  DifferentiatorOutMin=[]  DifferentiatorOutMax=[]  FilterDiffOutCoefMin=[]  FilterDiffOutCoefMax=[]  ReciprocalOutMin=[]  ReciprocalOutMax=[]  SumDenOutMin=[]  SumDenOutMax=[]  SumNumOutMin=[]  SumNumOutMax=[]  DivideOutMin=[]  DivideOutMax=[]  UdiffTsProdOutMin=[]  UdiffTsProdOutMax=[]  NTsProdOutMin=[]  NTsProdOutMax=[]  UintegralTsProdOutMin=[]  UintegralTsProdOutMax=[]  UngainTsProdOutMin=[]  UngainTsProdOutMax=[]  ClampingZeroOutDataTypeStr=Inherit: Inherit via back propagation  ClampingZeroOutMin=[]  ClampingZeroOutMax=[]  FilterDenConstantOutDataTypeStr=Inherit: Inherit via back propagation  FilterDenConstantOutMin=[]  FilterDenConstantOutMax=[]  PCopyOutDataTypeStr=Inherit: Inherit via back propagation  PCopyOutMin=[]  PCopyOutMax=[]  NCopyOutDataTypeStr=Inherit: Inherit via back propagation  NCopyOutMin=[]  NCopyOutMax=[]  IntegratorContinuousStateAttributes=''  IntegratorStateMustResolveToSignalObject=off  IntegratorRTWStateStorageClass=Auto  FilterContinuousStateAttributes=''  FilterStateMustResolveToSignalObject=off  FilterRTWStateStorageClass=Auto  ParallelPVariant=InternalParameters  IdealPVariant=Disabled  IVariant=InternalParameters  DVariant=InternalParameters  IntegratorVariant=Discrete  SatVariant=Enabled  AWVariant=DiscClampingParallel  PCopyVariant=Disabled  TRVariant=Disabled  FdbkBlocksVariant=Forward  IdealPFdbkVariant=Disabled  SatFdbkVariant=Disabled  DerivativeFilterVariant=ForwardEulerFilter  NVariant=InternalParameters  NCopyVariant=Disabled  FilterICVariant=InternalICsFilter  IntegratorICVariant=InternalICs  ExternalResetVariant=Disabled  TRSumVariant=Passthrough  SumFdbkVariant=Disabled  SumVariant=Sum_PID  TsampFilterVariant=InternalTs  TsampNgainVariant=Passthrough  TsampIntegralVariant=Disabled_SignalSpec  ExternalSaturationOutDataTypeStr=Inherit: Same as second input  DerivativeSourceVariant=ErrorSignal  PreIntVariant=InternalPreInt
  Sum : Sum  Inputs=|+-
  Tmax_rr : Outport  OutDataTypeStr=single  PortDimensions=1  SampleTime=0.003
  wires:
  PID Controller/1 -> Tmax_rr/1  "Tmax_rr_Nm"
  Sum/1 -> PID Controller/1  "e"
  kappa_rr/1 -> Sum/2  "kappa_rr"
  1-D Lookup Table/1 -> Sum/1  "kappa_ref"
  Fz_rr/1 -> 1-D Lookup Table/1  "Fz_rr_N"

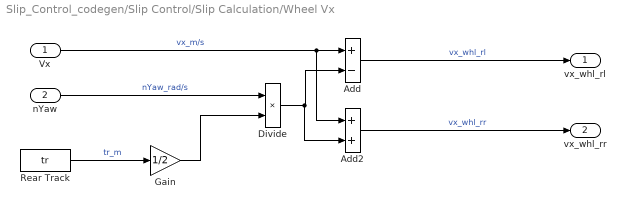
== system Slip_Control_codegen/Slip Control/Slip Calculation/Wheel Vx ==
  Vx : Inport  OutDataTypeStr=single  PortDimensions=1  SampleTime=0.003
  nYaw : Inport  Port=2  OutDataTypeStr=single  PortDimensions=1  SampleTime=0.003
  Add : Sum  Inputs=+-  OutDataTypeStr=single  AccumDataTypeStr=single
  Add2 : Sum  OutDataTypeStr=single  AccumDataTypeStr=single
  Divide : Product  Inputs=**  OutDataTypeStr=single
  Gain : Gain  Gain=1/2  ParamDataTypeStr=single  OutDataTypeStr=single
  Rear Track : Constant  Value=tr  OutDataTypeStr=single
  vx_whl_rl : Outport  OutDataTypeStr=single  PortDimensions=1  SampleTime=0.003
  vx_whl_rr : Outport  Port=2  OutDataTypeStr=single  PortDimensions=1  SampleTime=0.003
  wires:
  Add2/1 -> vx_whl_rr/1  "vx_whl_rr"
  Add/1 -> vx_whl_rl/1  "vx_whl_rl"
  Divide/1 -> Add/2, Add2/2
  Vx/1 -> Add/1, Add2/1  "vx_m/s"
  Gain/1 -> Divide/2
  nYaw/1 -> Divide/1  "nYaw_rad/s"
  Rear Track/1 -> Gain/1  "tr_m"
